simulink model "iterative_motion_controller"  (R2026a)
settings: Solver=FixedStepDiscrete  StopTime=1
undefined symbols (not defined in the file): Amcmj1InitConf, MAX_EVENTS_PER_TICK, N_MOTORS, Ts_ControlFOC
settings Model: DataDictionary=amcmj1.sldd  Creator=mfussi  LastModifiedBy=rpumpo
settings SolverCC: ConcurrentTasks=on  InsertRTBMode=Never (minimum delay)
settings OptimizationCC: GainParamInheritBuiltInType=on  UseFloatMulNetSlope=on  DefaultUnderspecifiedDataType=single  UseSpecifiedMinMax=on  InlineInvariantSignals=on  SimCompilerOptimization=on
settings HardwareCC: ProdLargestAtomicInteger=Long  ProdLargestAtomicFloat=Double  ProdHWDeviceType=ARM Compatible->ARM Cortex-M
settings ModelReferenceCC: EnableParallelModelReferenceBuilds=on  ModelReferenceNumInstancesAllowed=Single
settings RTWCC: SystemTargetFile=ert.tlc  GenCodeOnly=on  PackageGeneratedCodeAndArtifacts=on  GenerateReport=on  RTWUseSimCustomCode=on  BuildConfiguration=Faster Runs  LaunchReport=on  TargetLang=C++  GenerateCodeMetricsReport=on  GenerateCodeReplacementReport=on  Description=Embedded Coder
settings CodeAppCC: MaxIdLength=60.0
settings ERTTargetCC: RootIOFormat=Structure reference  DynamicArrayContainerType=coder::array  TargetLangStandard=C++03 (ISO)  CodeReplacementLibrary=iCubTech  CombineSignalStateStructs=on  SuppressErrorStatus=on  SupportNonFinite=off

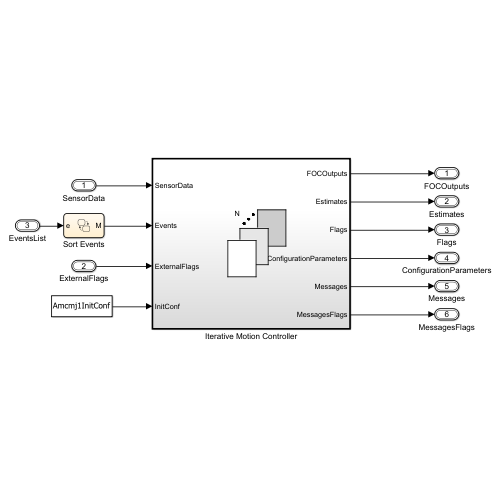
[thumbnail: Simulink's stored preview of the top-level diagram]
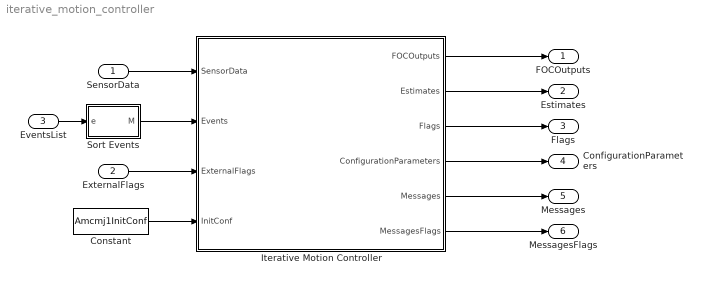
== system iterative_motion_controller ==
  SensorData : Inport  OutDataTypeStr=Bus: SensorsData  PortDimensions=N_MOTORS  SampleTime=Ts_ControlFOC  BusOutputAsStruct=on
  ExternalFlags : Inport  Port=2  OutDataTypeStr=Bus: ExternalFlags  BusOutputAsStruct=on
  EventsList : Inport  Port=3  OutDataTypeStr=Bus: ReceivedEvents  PortDimensions=N_MOTORS*MAX_EVENTS_PER_TICK  BusOutputAsStruct=on
  Constant : Constant  Value=Amcmj1InitConf  OutDataTypeStr=Bus: ActuatorConfiguration  SampleTime=1e-3
  Iterative Motion Controller : Subsystem  TreatAsAtomicUnit=on
  Sort Events : Stateflow chart  TreatAsAtomicUnit=on
  FOCOutputs : Outport  OutDataTypeStr=Bus: FOCOutputs  BusOutputAsStruct=on
  Estimates : Outport  Port=2  OutDataTypeStr=Bus: EstimatedData  BusOutputAsStruct=on
  Flags : Outport  Port=3  OutDataTypeStr=Bus: Flags  BusOutputAsStruct=on
  ConfigurationParameters : Outport  Port=4  OutDataTypeStr=Bus: ActuatorConfiguration  BusOutputAsStruct=on
  Messages : Outport  Port=5  OutDataTypeStr=Bus: BUS_MESSAGES_TX  BusOutputAsStruct=on
  MessagesFlags : Outport  Port=6  OutDataTypeStr=Bus: BUS_STATUS_TX  BusOutputAsStruct=on
  wires:
  EventsList/1 -> Sort Events/1(e)
  Iterative Motion Controller/3(Flags) -> Flags/1
  ExternalFlags/1 -> Iterative Motion Controller/3(ExternalFlags)
  Iterative Motion Controller/2(Estimates) -> Estimates/1
  Constant/1 -> Iterative Motion Controller/4(InitConf)
  Sort Events/1(M) -> Iterative Motion Controller/2(Events)
  SensorData/1 -> Iterative Motion Controller/1(SensorData)
  Iterative Motion Controller/5(Messages) -> Messages/1
  Iterative Motion Controller/1(FOCOutputs) -> FOCOutputs/1
  Iterative Motion Controller/4(ConfigurationParameters) -> ConfigurationParameters/1
  Iterative Motion Controller/6(MessagesFlags) -> MessagesFlags/1

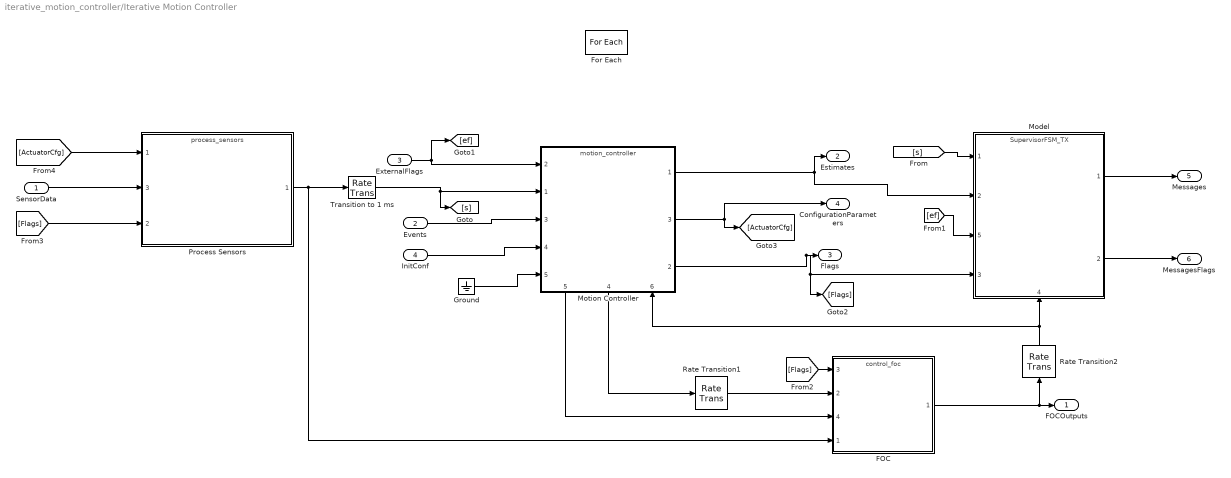
== system iterative_motion_controller/Iterative Motion Controller ==
  SensorData : Inport  OutDataTypeStr=Bus: SensorsData  Partition=on  PartitionDimension=1  PartitionWidth=1  PartitionOffset=0
  Events : Inport  Port=2  OutDataTypeStr=Bus:ReceivedEvents  Partition=on  PartitionDimension=1  PartitionWidth=1  PartitionOffset=0
  ExternalFlags : Inport  Port=3  OutDataTypeStr=Bus: ExternalFlags
  InitConf : Inport  Port=4  OutDataTypeStr=Bus: ActuatorConfiguration  Partition=on  PartitionDimension=1  PartitionWidth=1  PartitionOffset=0
  FOC : ModelReference  ModelNameDialog=control_foc.slx  ModelReferenceVersion=10.9
      settings: PortSchema="{\"entries\":[{\"content\":{\"sides\":[{\"content\":{\"connectorIds\":[\"In3\",\"In2\",\"In4\",\"In1\"]},\"type\":\"ConnectorPlacement.EquallySpacedRectSide\",\"uuid\":\"276821a8-1675-47c1-bf5c-bb820cdd6cd6\"},{\"content\":{\"connectorIds\":[\"Out1\"],\"side\":\"RIGHT\"},\"type\":\"ConnectorPlacement.EquallySpacedRectSide\",\"uuid\":\"2db17b86-a732-453f-8037-c6f8a66a9b4a\"},{\"content\":{\"side\":\"TOP\"},\"type\":\"ConnectorPlacement.EquallySpacedRectSide\",\"uuid\":\"c7644d9e-cb10-4f85-a70a-3c317f0edbe1\"}]},\"type\":\"ConnectorPlacement.EquallySpacedConnector\",\"uuid\":\"bebe9871-ce7e-40e5-8aa4-5c9db9197496\"}],\"packageUris\":[\"http://schema.mathworks.com/mf0/Connector/R2020b\"],\"version\":\"1.0\"}"
  For Each : ForEach  DisableCoverage=on
  Ground : Ground
  Model : ModelReference  ModelNameDialog=SupervisorFSM_TX.slx  ModelReferenceVersion=11.21
      settings: PortSchema="{\"entries\":[{\"content\":{\"sides\":[{\"content\":{\"connectorIds\":[\"In1\",\"In2\",\"In5\",\"In3\"]},\"type\":\"ConnectorPlacement.EquallySpacedRectSide\",\"uuid\":\"da3a0c31-d41a-44f2-85ec-d1033079ee97\"},{\"content\":{\"connectorIds\":[\"Out1\",\"Out2\"],\"side\":\"RIGHT\"},\"type\":\"ConnectorPlacement.EquallySpacedRectSide\",\"uuid\":\"20109ca7-306f-4d99-aef0-3fab938882d1\"},{\"content\":{\"side\":\"TOP\"},\"type\":\"ConnectorPlacement.EquallySpacedRectSide\",\"uuid\":\"7be952f9-d28b-4eac-8fc6-f95f374eaa80\"},{\"content\":{\"connectorIds\":[\"In4\"],\"side\":\"BOTTOM\"},\"type\":\"ConnectorPlacement.EquallySpacedRectSide\",\"uuid\":\"4258288d-da37-4e3f-a5e7-f71f9227c286\"}]},\"type\":\"ConnectorPlacement.EquallySpacedConnector\",\"uuid\":\"a950c446-ce16-41c8-9269-d83d512a5505\"}],\"packageUris\":[\"http://schema.mathworks.com/mf0/Connector/R2020b\"],\"version\":\"1.0\"}"
  Motion Controller : ModelReference  ModelNameDialog=motion_controller.slx  ModelReferenceVersion=6.15
      settings: PortSchema="{\"entries\":[{\"content\":{\"sides\":[{\"content\":{\"connectorIds\":[\"In2\",\"In1\",\"In3\",\"In4\",\"In5\"]},\"type\":\"ConnectorPlacement.EquallySpacedRectSide\",\"uuid\":\"e9b5b65c-955f-4ef8-87d2-abd1dc9c6b8f\"},{\"content\":{\"connectorIds\":[\"Out1\",\"Out3\",\"Out2\"],\"side\":\"RIGHT\"},\"type\":\"ConnectorPlacement.EquallySpacedRectSide\",\"uuid\":\"3af916ce-7ad5-4047-a735-392fad3d255a\"},{\"content\":{\"side\":\"TOP\"},\"type\":\"ConnectorPlacement.EquallySpacedRectSide\",\"uuid\":\"c9e16917-89aa-4334-8909-02234e79432d\"},{\"content\":{\"connectorIds\":[\"Out5\",\"Out4\",\"In6\"],\"side\":\"BOTTOM\"},\"type\":\"ConnectorPlacement.EquallySpacedRectSide\",\"uuid\":\"204d9c4a-11d0-49a3-86e6-b92f3b615404\"}]},\"type\":\"ConnectorPlacement.EquallySpacedConnector\",\"uuid\":\"a8c19507-f66d-439a-930b-5d4c4973b2d8\"}],\"packageUris\":[\"http://schema.mathworks.com/mf0/Connector/R2020b\"],\"version\":\"1.0\"}"
  Process Sensors : ModelReference  ModelNameDialog=process_sensors.slx  ModelReferenceVersion=2.1
      settings: PortSchema="{\"entries\":[{\"content\":{\"sides\":[{\"content\":{\"connectorIds\":[\"In1\",\"In3\",\"In2\"]},\"type\":\"ConnectorPlacement.EquallySpacedRectSide\",\"uuid\":\"abe329f5-3a6f-4f94-8a31-73b44f8729e1\"},{\"content\":{\"connectorIds\":[\"Out1\"],\"side\":\"RIGHT\"},\"type\":\"ConnectorPlacement.EquallySpacedRectSide\",\"uuid\":\"310f757e-124e-471f-8694-94a58df13cf5\"},{\"content\":{\"side\":\"TOP\"},\"type\":\"ConnectorPlacement.EquallySpacedRectSide\",\"uuid\":\"c5ed01f2-9990-4439-8db2-971f0d207839\"}]},\"type\":\"ConnectorPlacement.EquallySpacedConnector\",\"uuid\":\"f4b7f613-2a7b-45d0-9d52-9ca9a72a6394\"}],\"packageUris\":[\"http://schema.mathworks.com/mf0/Connector/R2020b\"],\"version\":\"1.0\"}"
  Rate Transition1 : RateTransition  Deterministic=off  OutPortSampleTime=Ts_ControlFOC
  Rate Transition2 : RateTransition  Deterministic=off  OutPortSampleTime=Ts_Supervision
  Transition to 1 ms : RateTransition  Deterministic=off  OutPortSampleTime=Ts_Supervision
  FOCOutputs : Outport  OutDataTypeStr=Bus: FOCOutputs  ConcatenationDimension=1
  Estimates : Outport  Port=2  OutDataTypeStr=Bus: EstimatedData  ConcatenationDimension=1
  Flags : Outport  Port=3  OutDataTypeStr=Bus: Flags  ConcatenationDimension=1
  ConfigurationParameters : Outport  Port=4  OutDataTypeStr=Bus: ActuatorConfiguration  ConcatenationDimension=1
  Messages : Outport  Port=5  ConcatenationDimension=1
  MessagesFlags : Outport  Port=6  ConcatenationDimension=1
  wires:
  ExternalFlags/1 -> Motion Controller/2, [ef]
  InitConf/1 -> Motion Controller/4
  Events/1 -> Motion Controller/3
  [s] -> Model/1
  [ef] -> Model/5
  Model/1 -> Messages/1
  Model/2 -> MessagesFlags/1
  Ground/1 -> Motion Controller/5
  Motion Controller/1 -> Estimates/1, Model/2
  Motion Controller/3 -> ConfigurationParameters/1, [ActuatorCfg]
  Transition to 1 ms/1 -> Motion Controller/1, [s]
  FOC/1 -> Rate Transition2/1, FOCOutputs/1
  Rate Transition2/1 -> Motion Controller/6, Model/4
  Motion Controller/2 -> [Flags], Model/3, Flags/1
  [Flags] -> FOC/3
  [Flags] -> Process Sensors/2
  [ActuatorCfg] -> Process Sensors/1
  Rate Transition1/1 -> FOC/2
  Motion Controller/4 -> Rate Transition1/1
  Motion Controller/5 -> FOC/4
  SensorData/1 -> Process Sensors/3
  Process Sensors/1 -> Transition to 1 ms/1, FOC/1

== stateflow chart iterative_motion_controller/Sort Events ==
  settings: initializeOutput=1
  (default) -> (junction 13) : % Bin Events
  (junction 13) -> (junction 15) : {idx = 0;
      | counter_motor_1 = 0;
      | counter_motor_2 = 0;}
  (junction 15) -> (junction 14) [order 1] : [idx < N_MOTORS*MAX_EVENTS_PER_TICK]
  (junction 14) -> (junction 60) [order 1] : [e[idx].motor_id == 0 && counter_motor_1 < MAX_EVENTS_PER_TICK]{
      | M[e[idx].motor_id][counter_motor_1] = e[idx];
      | counter_motor_1++;}
  (junction 14) -> (junction 61) [order 2] : [e[idx].motor_id == 1 && counter_motor_2 < MAX_EVENTS_PER_TICK]{
      | M[e[idx].motor_id][counter_motor_2 ] = e[idx];
      | counter_motor_2++;}
  (junction 17) -> (junction 15) : {idx++;}
  (junction 14) -> (junction 17) [order 3]
  (junction 60) -> (junction 61)
  (junction 15) -> (junction 59) [order 2]
  (junction 61) -> (junction 17)
  data: e input Bus: ReceivedEvents size=[N_MOTORS*MAX_EVENTS_PER_TICK]; M output Bus: ReceivedEvents size=[N_MOTORS, MAX_EVENTS_PER_TICK]; idx local uint8 size=1; counter_motor_1 local uint8 size=1; counter_motor_2 local uint8 size=1; MAX_EVENTS_PER_TICK parameter; N_MOTORS parameter
